simulink model "AOCS"  (R2026a)
settings: Solver=VariableStepAuto  StopTime=Tsim
InitFcn:
  | init
StopFcn:
  | plot_post
values from neighbouring files (symbols this model uses):
  b_rw = 0.0    (= 0)    [init.m]
  J_rw = 0.5 * mass_rw * (radius_rw^2)    (= 0.000245)    [init.m]
  J_sat = (1/12) * mass_sat * (width_sat^2 + height_sat^2)    (= 0.0291666666667)    [init.m]
settings Model: Creator=sayoo  LastModifiedBy=sayoo

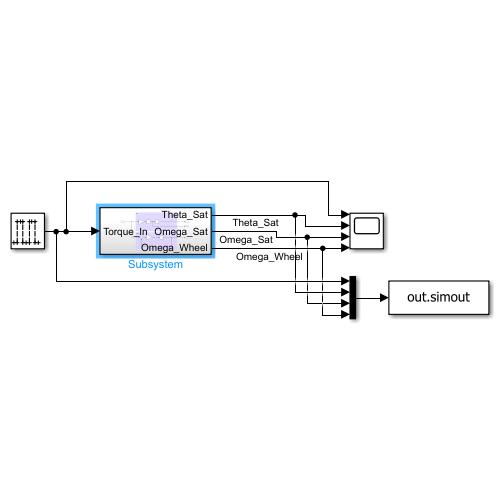
[thumbnail: Simulink's stored preview of the top-level diagram]
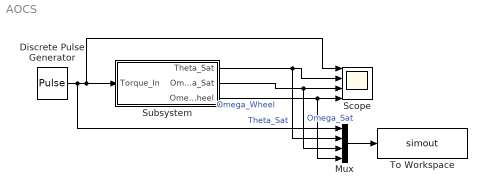
== system AOCS ==
  Discrete Pulse Generator : DiscretePulseGenerator  Amplitude=0.002  Period=20  PulseWidth=10  PhaseDelay=2
  Mux : Mux
  Scope : Scope  NumInputPorts=4
      settings: ActiveDisplayYMinimum=-52.110364479261264  ActiveDisplayYMaximum=135.08853958218467
  Subsystem : Subsystem
  To Workspace : ToWorkspace  VariableName=simout  SaveFormat=Timeseries  SampleTime=-1
  wires:
  Discrete Pulse Generator/1 -> Mux/1, Scope/1, Subsystem/1(Torque_In)
  Subsystem/1(Theta_Sat) -> Mux/2, Scope/2  "Theta_Sat"
  Subsystem/2(Omega_Sat) -> Mux/3, Scope/3  "Omega_Sat"
  Subsystem/3(Omega_Wheel) -> Mux/4, Scope/4  "Omega_Wheel"
  Mux/1 -> To Workspace/1

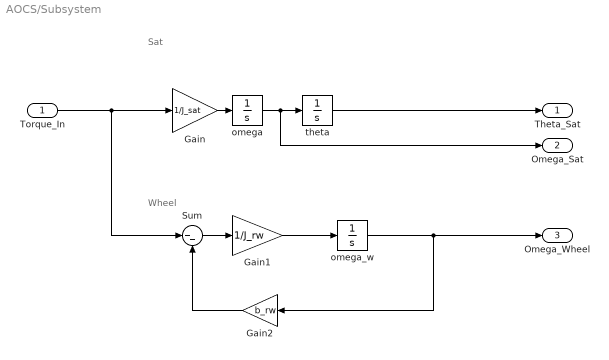
== system AOCS/Subsystem ==
  note: Sat
  note: Wheel
  Torque_In : Inport
  Gain : Gain  Gain=1/J_sat
  Gain1 : Gain  Gain=1/J_rw
  Gain2 : Gain  Gain=b_rw
  Sum : Sum  Inputs=|--
  omega : Integrator
  omega_w : Integrator
  theta : Integrator
  Theta_Sat : Outport
  Omega_Sat : Outport  Port=2
  Omega_Wheel : Outport  Port=3
  wires:
  Torque_In/1 -> Sum/1, Gain/1
  Gain/1 -> omega/1
  omega/1 -> Omega_Sat/1, theta/1
  theta/1 -> Theta_Sat/1
  Sum/1 -> Gain1/1
  Gain1/1 -> omega_w/1
  omega_w/1 -> Omega_Wheel/1, Gain2/1
  Gain2/1 -> Sum/2
